simulink model "IEEE13_DVR_DSTATCOM_PV_Wind"  (R2022a)
settings: Solver=ode4  StartTime=0.0  StopTime=1.0  FixedStep=Ts  MaxStep=1e-4  RelTol=1e-4
InitFcn:
  | a=1; % Loading Factor
  | Ts=50e-6;
  | % phase to sequence conversion of RXB matrices
  | c=1*exp(sqrt(-1)*(120*pi/180));
  | T=[1 1 1;1 c*c c;1 c c*c];
  | Tinv=1/3*[1 1 1;1 c c*c;1 c*c c];
  | 
  | % Simulation data for the IEEE 13 Node Test Feeder model
  | mi2km = 1.60934;%  miles to km conversion
  | ft2km = 0.0003048; % feet to km conversion
  | ms2F = 1*1e-6/(2*pi*60);% microsiemens to Farads conversion
  | 
  | 
  | %% Configuration 601
  | % Series Resitance and Reactance - ohm/mile
  | R_601 = [0.3465 0.1560 0.1580;0.1560 0.3375 0.1535;0.1580 0.1535 0.3414];
  | X_601 = [1.1079 0.5017 0.4236;0.5017 1.0478 0.3849;0.4236 0.3849 1.0348];
  | % charging susceptance - microsiemens/mile
  | B_601 = [6.2998 -1.9958 -1.2595;-1.9958 5.9597 -0.7417;-1.2595 -0.7417 5.6386];
  | 
  | R_601 = R_601/mi2km;
  | Rseq=Tinv*R_601*T;
  | R1_601=Rseq(2,2);R0_601=Rseq(1,1);
  | 
  | L_601 = (X_601/(2*pi*60))/mi2km;
  | Lseq=Tinv*L_601*T;
  | L1_601=Lseq(2,2);L0_601=Lseq(1,1);
  | 
  | C_601 =(B_601*ms2F)/mi2km;
  | Cseq=Tinv*C_601*T;
  | C1_601=Cseq(2,2);C0_601=Cseq(1,1);
  | 
  | %% Configuration 602 - series reactance - ohm/mile
  | R_602 = [0.7526 0.1580 0.1560;0.1580 0.7475 0.1535;0.1560 0.1535 0.7436];
  | X_602 = [1.1814 0.4236 0.5017;0.4236 1.1983 0.3849;0.5017 0.3849 1.2112];
  | % charging susceptance - microsiemens/mile
  | B_602 = [5.6990 -1.0817 -1.6905;-1.0817 5.1795 -0.6588;-1.6905 -0.6588 5.4246];
  | 
  | R_602 = R_602/mi2km;
  | Rseq=Tinv*R_602*T;
  | R1_602=Rseq(2,2);R0_602=Rseq(1,1);
  | 
  | L_602 = (X_602/(2*pi*60))/mi2km;
  | Lseq=Tinv*L_602*T;
  | L1_602=Lseq(2,2);L0_602=Lseq(1,1);
  | 
  | C_602 =(B_602*ms2F)/mi2km;
  | Cseq=Tinv*C_602*T;
  | C1_602=Cseq(2,2);C0_602=Cseq(1,1);
  | %% Configuration 603 - series reactance - ohm/mile
  | R_603 = [0 0 0;0 1.3294 0.2066;0 0.2066 1.3238];
  | X_603 = [0 0 0;0 1.3471 0.4591;0 0.4591 1.3569];
  | % charging susceptance - microsiemens/mile
  | B_603 = [0 0 0;0 4.7097 -0.8999;0 -0.8999 4.6658];
  | 
  | % convert for SPS
  | R_603 = R_603/mi2km;
  | Rseq=Tinv*R_603*T;
  | R1_603=Rseq(2,2);R0_603=Rseq(1,1);
  | 
  | ... (+71 lines)
undefined symbols (not defined in the file): find_system
libraries: spsGroundLib x48, spsSeriesRLCBranchLib x46, spsThreePhaseVIMeasurementLib x19, spsControlledVoltageSourceLib x15, spsThreePhaseSeriesRLCLoadLib x7, spsRMSLib x7, spsThreePhaseBreakerLib x6, spsVoltageMeasurementLib x6, spsOnDelayLib x6, spsThreePhasePISectionLineLib x5, spsSeriesRLCLoadLib x5, spsMutualInductanceLib x4
(part 2 of 4)

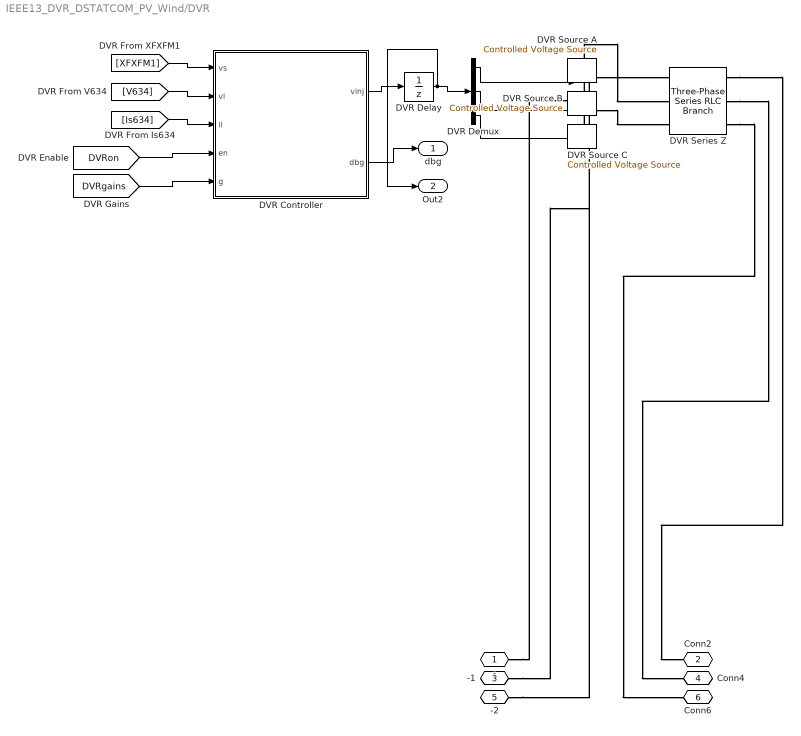
== system IEEE13_DVR_DSTATCOM_PV_Wind/DVR ==
  DVR Controller : MATLAB Function  TreatAsAtomicUnit=on
  DVR Delay : UnitDelay  SampleTime=-1  HasFrameUpgradeWarning=on
  DVR Demux : Demux  Outputs=3
  DVR Series Z : spsThreePhaseSeriesRLCBranchLib/Three-Phase Series RLC Branch  LConnTagsString=A|B|C  RConnTagsString=A|B|C  BranchType=RL  Resistance=2e-3  Inductance=60e-6  Capacitance=1e-6  Measurements=None
  DVR Source A : spsControlledVoltageSourceLib/Controlled Voltage Source  Initialize=off  Source_Type=AC  Amplitude=0  Phase=0  Frequency=0  Measurements=None
  DVR Source B : spsControlledVoltageSourceLib/Controlled Voltage Source  Initialize=off  Source_Type=AC  Amplitude=0  Phase=0  Frequency=0  Measurements=None
  DVR Source C : spsControlledVoltageSourceLib/Controlled Voltage Source  Initialize=off  Source_Type=AC  Amplitude=0  Phase=0  Frequency=0  Measurements=None
  - : PMIOPort  Side=Left
  Conn2 : PMIOPort  Port=2  Side=Right
  -1 : PMIOPort  Port=3  Side=Left
  Conn4 : PMIOPort  Port=4  Side=Right
  -2 : PMIOPort  Port=5  Side=Left
  Conn6 : PMIOPort  Port=6  Side=Right
  dbg : Outport
  Out2 : Outport  Port=2
  wires:
  DVR Demux/3 -> DVR Source C/1
  DVR Controller/1(vinj) -> DVR Delay/1
  DVR Delay/1 -> Out2/1, DVR Demux/1
  DVR Demux/2 -> DVR Source B/1
  [Is634] -> DVR Controller/3(il)
  [XFXFM1] -> DVR Controller/1(vs)
  DVR Demux/1 -> DVR Source A/1
  [V634] -> DVR Controller/2(vl)
  DVR Controller/2(dbg) -> dbg/1
  [DVRon] -> DVR Controller/4(en)
  [DVRgains] -> DVR Controller/5(g)
  connections:
  DVR Series Z/RConn2 -- Conn4/RConn1
  -2/RConn1 -- DVR Source C/LConn1
  DVR Series Z/RConn1 -- Conn2/RConn1
  DVR Source A/RConn1 -- DVR Series Z/LConn1
  DVR Source B/RConn1 -- DVR Series Z/LConn2
  DVR Source C/RConn1 -- DVR Series Z/LConn3
  -1/RConn1 -- DVR Source B/LConn1
  -/RConn1 -- DVR Source A/LConn1
  DVR Series Z/RConn3 -- Conn6/RConn1

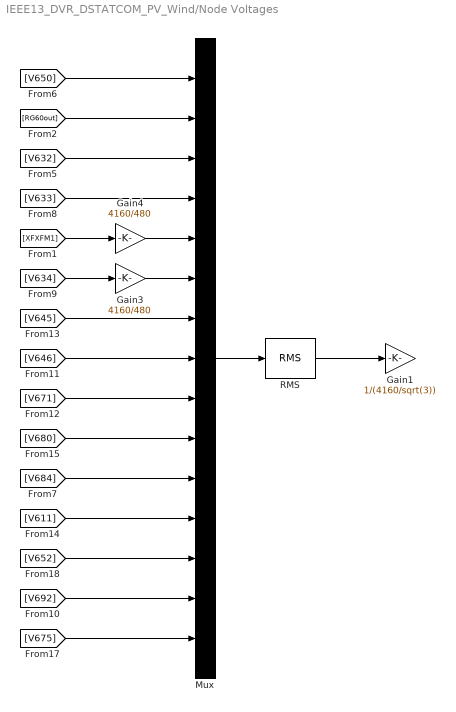
== system IEEE13_DVR_DSTATCOM_PV_Wind/Node Voltages ==
  Gain1 : Gain  Gain=1/(4160/sqrt(3))
  Gain3 : Gain  Gain=4160/480
  Gain4 : Gain  Gain=4160/480
  Mux : Mux  Inputs=15
  RMS : spsRMSLib/RMS  TrueRMS=on  Freq=60  RMSInit=120  Ts=0
  wires:
  RMS/1 -> Gain1/1
  Mux/1 -> RMS/1
  [V634] -> Gain3/1
  [V684] -> Mux/11
  [V675] -> Mux/15
  [V646] -> Mux/8
  [V633] -> Mux/4
  Gain3/1 -> Mux/6
  [XFXFM1] -> Gain4/1
  [V611] -> Mux/12
  [V632] -> Mux/3
  [V671] -> Mux/9
  [V680] -> Mux/10
  [V650] -> Mux/1
  [V652] -> Mux/13
  [RG60out] -> Mux/2
  [V692] -> Mux/14
  [V645] -> Mux/7
  Gain4/1 -> Mux/5

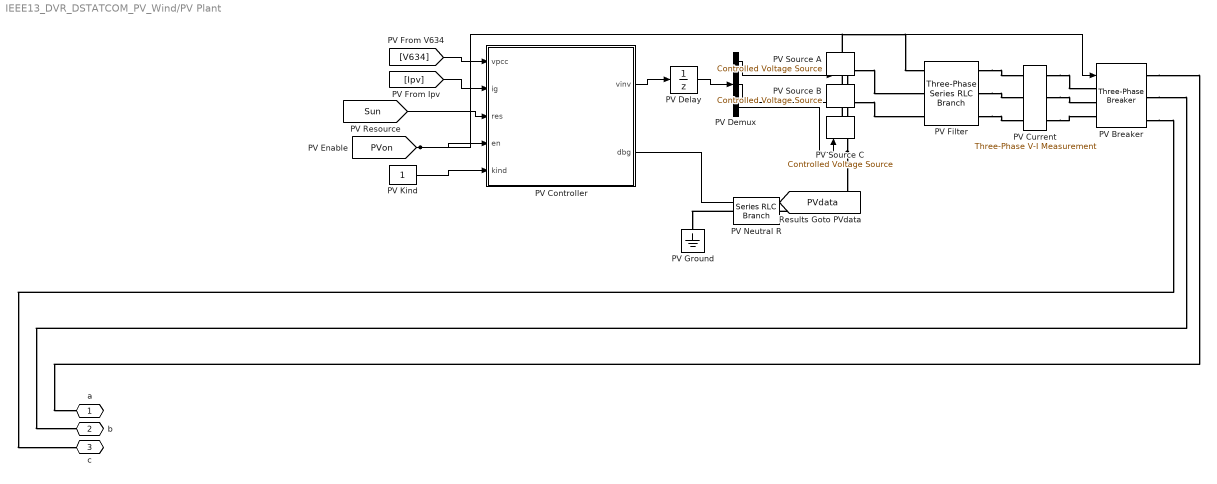
== system IEEE13_DVR_DSTATCOM_PV_Wind/PV Plant ==
  PV Breaker : spsThreePhaseBreakerLib/Three-Phase Breaker  InitialState=open  SwitchA=on  SwitchB=on  SwitchC=on  SwitchTimes=[0.2]  External=on  BreakerResistance=0.01  SnubberResistance=1e6  SnubberCapacitance=inf  Measurements=None
  PV Controller : MATLAB Function  TreatAsAtomicUnit=on
  PV Current : spsThreePhaseVIMeasurementLib/Three-Phase V-I Measurement  VoltageMeasurement=no  SetLabelV=off  LabelV=Vabc  Vpu=off  VpuLL=off  CurrentMeasurement=yes  SetLabelI=on  LabelI=Ipv  Ipu=off  Pbase=100e6  Vbase=500e3  OutputType=Complex  PhasorSimulation=off  PSBequivalent=0
  PV Delay : UnitDelay  SampleTime=-1  HasFrameUpgradeWarning=on
  PV Demux : Demux  Outputs=3
  PV Filter : spsThreePhaseSeriesRLCBranchLib/Three-Phase Series RLC Branch  LConnTagsString=A|B|C  RConnTagsString=A|B|C  BranchType=RL  Resistance=0.01*480^2/450e3  Inductance=0.1*480^2/450e3/(2*pi*60)  Capacitance=1e-6  Measurements=None
  PV Ground : spsGroundLib/Ground  LConnTagsString=a
  PV Kind : Constant  SampleTime=50e-6
  PV Neutral R : spsSeriesRLCBranchLib/Series RLC Branch  LConnTagsString=__new0  RConnTagsString=__new0  BranchType=R  Resistance=1e6  Inductance=1e-3  SetiL0=off  InitialCurrent=0  Capacitance=1e-6  Setx0=off  InitialVoltage=0  Measurements=None
  PV Source A : spsControlledVoltageSourceLib/Controlled Voltage Source  Initialize=off  Source_Type=AC  Amplitude=0  Phase=0  Frequency=0  Measurements=None
  PV Source B : spsControlledVoltageSourceLib/Controlled Voltage Source  Initialize=off  Source_Type=AC  Amplitude=0  Phase=0  Frequency=0  Measurements=None
  PV Source C : spsControlledVoltageSourceLib/Controlled Voltage Source  Initialize=off  Source_Type=AC  Amplitude=0  Phase=0  Frequency=0  Measurements=None
  a : PMIOPort  Side=Right
  b : PMIOPort  Port=2  Side=Right
  c : PMIOPort  Port=3  Side=Right
  tag scope: PVdata=global
  wires:
  [V634] -> PV Controller/1(vpcc)
  [Ipv] -> PV Controller/2(ig)
  PV Delay/1 -> PV Demux/1
  PV Kind/1 -> PV Controller/5(kind)
  PV Controller/2(dbg) -> [PVdata]
  PV Controller/1(vinv) -> PV Delay/1
  PV Demux/1 -> PV Source A/1
  PV Demux/3 -> PV Source C/1
  PV Demux/2 -> PV Source B/1
  [PVon] -> PV Controller/4(en), PV Breaker/1
  [Sun] -> PV Controller/3(res)
  connections:
  PV Source A/LConn1 -- PV Neutral R/RConn1 -- PV Source C/LConn1 -- PV Source B/LConn1
  PV Neutral R/LConn1 -- PV Ground/LConn1
  PV Filter/RConn1 -- PV Current/LConn1
  PV Source B/RConn1 -- PV Filter/LConn2
  PV Source C/RConn1 -- PV Filter/LConn3
  PV Filter/RConn2 -- PV Current/LConn2
  PV Filter/RConn3 -- PV Current/LConn3
  PV Current/RConn3 -- PV Breaker/LConn3
  PV Source A/RConn1 -- PV Filter/LConn1
  PV Current/RConn1 -- PV Breaker/LConn1
  PV Current/RConn2 -- PV Breaker/LConn2
  PV Breaker/RConn1 -- a/RConn1
  PV Breaker/RConn3 -- c/RConn1
  PV Breaker/RConn2 -- b/RConn1

== system IEEE13_DVR_DSTATCOM_PV_Wind/Regulator 1 ==
  Mux : Mux  Inputs=3
  Single Phase SVR_A : Subsystem  LoadFcn=find_system(gcs,'FollowLinks', 'on', 'LookUnderMasks', 'all');  mask(Single-Phase OLTC){pNom=5e6/3, fNom=60, vNom=4160/sqrt(3), ctRatio=700, ptRatio=20, DeltaU=0.00625, TapMinMax=[-16 16], InitialTap=-10, TapSelectionTime=0.2, RegulatorOn=on, Regulator=[122/120  2/120  0.2], Comp=[3 9]}
      mask prompts: pNom "Nominal Power (VA)"; fNom "Nominal Frequency (Hz)"; vNom "Nominal Voltage (Vrms)"; ctRatio "Primary CT Rating (A)"; ptRatio "PT Ratio"; DeltaU "Voltage Step Per Tap (pu)"; TapMinMax "Minimum and Maximum Tap Positions"; InitialTap "Initial Tap Position"; TapSelectionTime "Tap Selection Time (s)"; RegulatorOn "Voltage Regulator"; Regulator "Voltage Regulator [ Vref(pu) DeadBand(pu)  Delay(s)]"; Comp "Compensator Settings [R (V) X(V)]"
      mask help:
      | Models a single-phase On Load Tap Changer (OLTC). The single-phase primary of multi-tap winding is modeled with a Variable-Ratio Transformer block.
      |
      | The transformer voltage ratio U2/U1 (in pu) is given by:
      |                 U2/U1= 1/ (1+TapPosition*DeltaU)
      | Tap position 0 corresponds to nominal voltage ratio.
      |
      | When Voltage regulator is 'on',  voltage regulator asks for a tap change if:
      |                  abs(Vm-Vref)>DeadBand/2  during a time  t > Delay.
      |
      | where 'Vm' is voltage measured at regulating point and Vref is reference voltage.
      | With line drop compensation, Vm=Vsec-Isec(R+jX)
      mask init:
      | RegulatorVref=Regulator(1);
      | RegulatorDeadBand=Regulator(2);
      | RegulatorDelay=Regulator(3);
      | Rc=Comp(1);
      | Xc=Comp(2);
      mask TypeOptions RegulatorOn: off | on
      mask Callback RegulatorOn:
      | tempMaskVis=get_param(gcb,'MaskVisibilities');
      | if strcmp(get_param(gcb,'RegulatorOn'),'on')
      | 	tempMaskVis{11}='on';
      | 	set_param(gcb,'MaskVisibilities',tempMaskVis);
      | else
      | 	tempMaskVis{11}='off';
      | 	set_param(gcb,'MaskVisibilities',tempMaskVis);
      | end
      | if strcmp(get_param(gcb,'RegulatorOn'),'on')
      | 	tempMaskVis{12}='on';
      | 	set_param(gcb,'MaskVisibilities',tempMaskVis);
      | else
      | 	tempMaskVis{12}='off';
      | 	set_param(gcb,'MaskVisibilities',tempMaskVis);
      | end
      mask DialogControl Container8 Prompt: Setup
      mask DialogControl Container13 Prompt: Regulator Parameters
      mask Display:
      | color('blue');
      | r=50;x=40;y=80;
      | th = 0:pi/100:2*pi;
      | f = r * exp(j*th) + x+j*y;
      | plot(real(f), imag(f));
      | color('red');
      | plot([-10 90],[30,130])
      | plot([75 90],[125,130])
      | plot([85 90],[115,130])
      | color('black')
      | port_label('Lconn',1,'S');port_label('Rconn',1,'L');
  Single Phase SVR_B : Subsystem  LoadFcn=find_system(gcs,'FollowLinks', 'on', 'LookUnderMasks', 'all');  mask(Single-Phase OLTC){pNom=5e6/3, fNom=60, vNom=4160/sqrt(3), ctRatio=700, ptRatio=20, DeltaU=0.00625, TapMinMax=[-16 16], InitialTap=-8, TapSelectionTime=0.2, RegulatorOn=on, Regulator=[122/120  2/120  0.2], Comp=[3 9]}
      mask prompts: pNom "Nominal Power (VA)"; fNom "Nominal Frequency (Hz)"; vNom "Nominal Voltage (Vrms)"; ctRatio "Primary CT Rating (A)"; ptRatio "PT Ratio"; DeltaU "Voltage Step Per Tap (pu)"; TapMinMax "Minimum and Maximum Tap Positions"; InitialTap "Initial Tap Position"; TapSelectionTime "Tap Selection Time (s)"; RegulatorOn "Voltage Regulator"; Regulator "Voltage Regulator [ Vref(pu) DeadBand(pu)  Delay(s)]"; Comp "Compensator Settings [R (V) X(V)]"
      mask help:
      | Models a single-phase On Load Tap Changer (OLTC). The single-phase primary of multi-tap winding is modeled with a Variable-Ratio Transformer block.
      |
      | The transformer voltage ratio U2/U1 (in pu) is given by:
      |                 U2/U1= 1/ (1+TapPosition*DeltaU)
      | Tap position 0 corresponds to nominal voltage ratio.
      |
      | When Voltage regulator is 'on',  voltage regulator asks for a tap change if:
      |                  abs(Vm-Vref)>DeadBand/2  during a time  t > Delay.
      |
      | where 'Vm' is voltage measured at regulating point and Vref is reference voltage.
      | With line drop compensation, Vm=Vsec-Isec(R+jX)
      mask init:
      | RegulatorVref=Regulator(1);
      | RegulatorDeadBand=Regulator(2);
      | RegulatorDelay=Regulator(3);
      | Rc=Comp(1);
      | Xc=Comp(2);
      mask TypeOptions RegulatorOn: off | on
      mask Callback RegulatorOn:
      | tempMaskVis=get_param(gcb,'MaskVisibilities');
      | if strcmp(get_param(gcb,'RegulatorOn'),'on')
      | 	tempMaskVis{11}='on';
      | 	set_param(gcb,'MaskVisibilities',tempMaskVis);
      | else
      | 	tempMaskVis{11}='off';
      | 	set_param(gcb,'MaskVisibilities',tempMaskVis);
      | end
      | if strcmp(get_param(gcb,'RegulatorOn'),'on')
      | 	tempMaskVis{12}='on';
      | 	set_param(gcb,'MaskVisibilities',tempMaskVis);
      | else
      | 	tempMaskVis{12}='off';
      | 	set_param(gcb,'MaskVisibilities',tempMaskVis);
      | end
      mask DialogControl Container8 Prompt: Setup
      mask DialogControl Container13 Prompt: Regulator Parameters
      mask Display:
      | color('blue');
      | r=50;x=40;y=80;
      | th = 0:pi/100:2*pi;
      | f = r * exp(j*th) + x+j*y;
      | plot(real(f), imag(f));
      | color('red');
      | plot([-10 90],[30,130])
      | plot([75 90],[125,130])
      | plot([85 90],[115,130])
      | color('black')
      | port_label('Lconn',1,'S');port_label('Rconn',1,'L');
  Single Phase SVR_C : Subsystem  LoadFcn=find_system(gcs,'FollowLinks', 'on', 'LookUnderMasks', 'all');  mask(Single-Phase OLTC){pNom=5e6/3, fNom=60, vNom=4160/sqrt(3), ctRatio=700, ptRatio=20, DeltaU=0.00625, TapMinMax=[-16 16], InitialTap=-11, TapSelectionTime=0.2, RegulatorOn=on, Regulator=[122/120  2/120  0.2], Comp=[3 9]}
      mask prompts: pNom "Nominal Power (VA)"; fNom "Nominal Frequency (Hz)"; vNom "Nominal Voltage (Vrms)"; ctRatio "Primary CT Rating (A)"; ptRatio "PT Ratio"; DeltaU "Voltage Step Per Tap (pu)"; TapMinMax "Minimum and Maximum Tap Positions"; InitialTap "Initial Tap Position"; TapSelectionTime "Tap Selection Time (s)"; RegulatorOn "Voltage Regulator"; Regulator "Voltage Regulator [ Vref(pu) DeadBand(pu)  Delay(s)]"; Comp "Compensator Settings [R (V) X(V)]"
      mask help:
      | Models a single-phase On Load Tap Changer (OLTC). The single-phase primary of multi-tap winding is modeled with a Variable-Ratio Transformer block.
      |
      | The transformer voltage ratio U2/U1 (in pu) is given by:
      |                 U2/U1= 1/ (1+TapPosition*DeltaU)
      | Tap position 0 corresponds to nominal voltage ratio.
      |
      | When Voltage regulator is 'on',  voltage regulator asks for a tap change if:
      |                  abs(Vm-Vref)>DeadBand/2  during a time  t > Delay.
      |
      | where 'Vm' is voltage measured at regulating point and Vref is reference voltage.
      | With line drop compensation, Vm=Vsec-Isec(R+jX)
      mask init:
      | RegulatorVref=Regulator(1);
      | RegulatorDeadBand=Regulator(2);
      | RegulatorDelay=Regulator(3);
      | Rc=Comp(1);
      | Xc=Comp(2);
      mask TypeOptions RegulatorOn: off | on
      mask Callback RegulatorOn:
      | tempMaskVis=get_param(gcb,'MaskVisibilities');
      | if strcmp(get_param(gcb,'RegulatorOn'),'on')
      | 	tempMaskVis{11}='on';
      | 	set_param(gcb,'MaskVisibilities',tempMaskVis);
      | else
      | 	tempMaskVis{11}='off';
      | 	set_param(gcb,'MaskVisibilities',tempMaskVis);
      | end
      | if strcmp(get_param(gcb,'RegulatorOn'),'on')
      | 	tempMaskVis{12}='on';
      | 	set_param(gcb,'MaskVisibilities',tempMaskVis);
      | else
      | 	tempMaskVis{12}='off';
      | 	set_param(gcb,'MaskVisibilities',tempMaskVis);
      | end
      mask DialogControl Container8 Prompt: Setup
      mask DialogControl Container13 Prompt: Regulator Parameters
      mask Display:
      | color('blue');
      | r=50;x=40;y=80;
      | th = 0:pi/100:2*pi;
      | f = r * exp(j*th) + x+j*y;
      | plot(real(f), imag(f));
      | color('red');
      | plot([-10 90],[30,130])
      | plot([75 90],[125,130])
      | plot([85 90],[115,130])
      | color('black')
      | port_label('Lconn',1,'S');port_label('Rconn',1,'L');
  A : PMIOPort  Side=Left
  a : PMIOPort  Port=2  Side=Right
  B : PMIOPort  Port=3  Side=Left
  b : PMIOPort  Port=4  Side=Right
  C : PMIOPort  Port=5  Side=Left
  c : PMIOPort  Port=6  Side=Right
  Tap : Outport
  wires:
  Mux/1 -> Tap/1
  Single Phase SVR_C/1(Tap) -> Mux/3
  Single Phase SVR_B/1(Tap) -> Mux/2
  Single Phase SVR_A/1(Tap) -> Mux/1
  connections:
  Single Phase SVR_C/RConn1 -- c/RConn1
  Single Phase SVR_C/LConn1 -- C/RConn1
  Single Phase SVR_B/RConn1 -- b/RConn1
  Single Phase SVR_B/LConn1 -- B/RConn1
  Single Phase SVR_A/LConn1 -- A/RConn1
  Single Phase SVR_A/RConn1 -- a/RConn1

== system IEEE13_DVR_DSTATCOM_PV_Wind/Regulator Taps  ==
  note: Here the taps of the Voltage Regulator are on primary side of transformers unlike in Benchmark document where taps are considered on secondary of transformer. Therefore the values used are negative of what is used in Benchmark document. Also the direction of Tap Operation will be in opposite direction as compared to Regulator having taps on secondary side of transformer.
  Band Width : Constant  Value=2
  Band Width1 : Constant  Value=2
  Gain : Gain  Gain=1/2
  Gain2 : Gain  Gain=1/2
  Scope3 : Scope  NumInputPorts=5
  Sum : Sum  Inputs=|++
  Sum1 : Sum  Inputs=|+-
  Tap : Scope
  Vref : Constant  Value=122
  Vref1 : Constant  Value=122
  wires:
  [Rg1] -> Tap/1
  Vref/1 -> Sum/1
  Band Width/1 -> Gain/1
  Gain/1 -> Sum/2
  Gain2/1 -> Sum1/2
  Band Width1/1 -> Gain2/1
  Vref1/1 -> Sum1/1
  Sum/1 -> Scope3/1  "Upper Limit"
  [Vr1a] -> Scope3/2  "Vra"
  [Vr1b] -> Scope3/3  "Vrb"
  [Vr1c] -> Scope3/4  "Vrc"
  Sum1/1 -> Scope3/5  "Lower Limit"

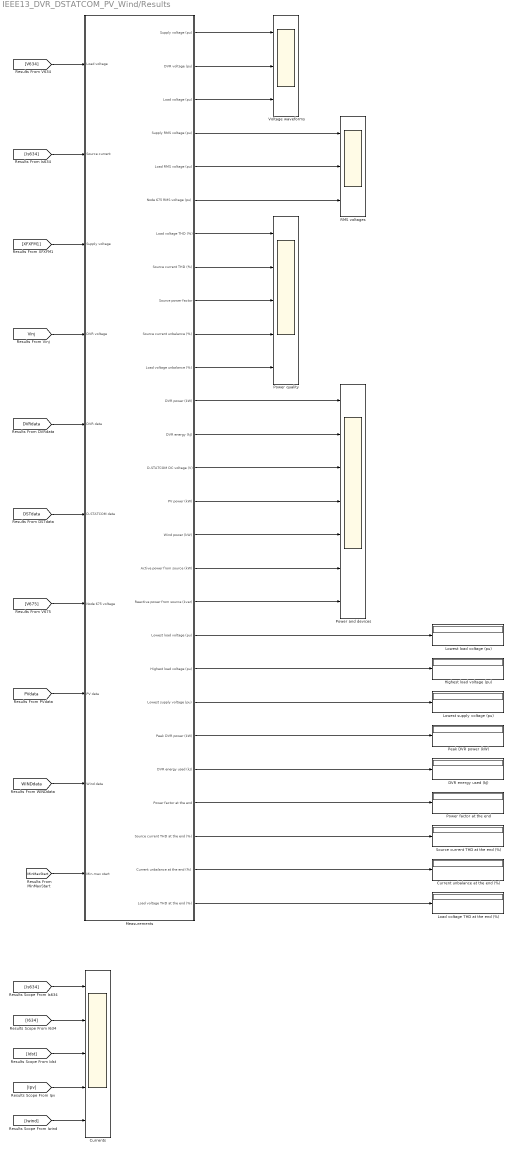
== system IEEE13_DVR_DSTATCOM_PV_Wind/Results ==
  Current unbalance at the end (%) : Display
      settings: Tag=results_panel
  Currents : Scope  NumInputPorts=5
      settings: Tag=results_panel
  DVR energy used (kJ) : Display
      settings: Tag=results_panel
  Highest load voltage (pu) : Display
      settings: Tag=results_panel
  Load voltage THD at the end (%) : Display
      settings: Tag=results_panel
  Lowest load voltage (pu) : Display
      settings: Tag=results_panel
  Lowest supply voltage (pu) : Display
      settings: Tag=results_panel
  Measurements : Subsystem  Tag=results_panel
  Peak DVR power (kW) : Display
      settings: Tag=results_panel
  Power and devices : Scope  NumInputPorts=7
      settings: Tag=results_panel
  Power factor at the end : Display
      settings: Tag=results_panel
  Power quality : Scope  NumInputPorts=5
      settings: Tag=results_panel
  RMS voltages : Scope  NumInputPorts=3
      settings: Tag=results_panel
  Source current THD at the end (%) : Display
      settings: Tag=results_panel
  Voltage waveforms : Scope  NumInputPorts=3
      settings: Tag=results_panel
  wires:
  Measurements/22(Peak DVR power (kW)) -> Peak DVR power (kW)/1
  [Idst] -> Currents/3
  Measurements/10(Source current unbalance (%)) -> Power quality/4
  [Is634] -> Currents/1
  Measurements/3(Load voltage (pu)) -> Voltage waveforms/3
  Measurements/19(Lowest load voltage (pu)) -> Lowest load voltage (pu)/1
  [WINDdata] -> Measurements/9(Wind data)
  Measurements/27(Load voltage THD at the end (%)) -> Load voltage THD at the end (%)/1
  Measurements/26(Current unbalance at the end (%)) -> Current unbalance at the end (%)/1
  [I634] -> Currents/2
  Measurements/2(DVR voltage (pu)) -> Voltage waveforms/2
  Measurements/14(D-STATCOM DC voltage (V)) -> Power and devices/3
  Measurements/16(Wind power (kW)) -> Power and devices/5
  Measurements/11(Load voltage unbalance (%)) -> Power quality/5
  Measurements/25(Source current THD at the end (%)) -> Source current THD at the end (%)/1
  [Vinj] -> Measurements/4(DVR voltage)
  Measurements/4(Supply RMS voltage (pu)) -> RMS voltages/1
  Measurements/13(DVR energy (kJ)) -> Power and devices/2
  Measurements/12(DVR power (kW)) -> Power and devices/1
  Measurements/24(Power factor at the end) -> Power factor at the end/1
  [Ipv] -> Currents/4
  Measurements/8(Source current THD (%)) -> Power quality/2
  Measurements/7(Load voltage THD (%)) -> Power quality/1
  Measurements/18(Reactive power from source (kvar)) -> Power and devices/7
  Measurements/20(Highest load voltage (pu)) -> Highest load voltage (pu)/1
  Measurements/6(Node 675 RMS voltage (pu)) -> RMS voltages/3
  Measurements/15(PV power (kW)) -> Power and devices/4
  Measurements/23(DVR energy used (kJ)) -> DVR energy used (kJ)/1
  [DVRdata] -> Measurements/5(DVR data)
  [Iwind] -> Currents/5
  Measurements/21(Lowest supply voltage (pu)) -> Lowest supply voltage (pu)/1
  Measurements/17(Active power from source (kW)) -> Power and devices/6
  Measurements/9(Source power factor) -> Power quality/3
  [Is634] -> Measurements/2(Source current)
  [PVdata] -> Measurements/8(PV data)
  Measurements/1(Supply voltage (pu)) -> Voltage waveforms/1
  [V675] -> Measurements/7(Node 675 voltage)
  Measurements/5(Load RMS voltage (pu)) -> RMS voltages/2
  [V634] -> Measurements/1(Load voltage)
  [DSTdata] -> Measurements/6(D-STATCOM data)
  [MinMaxStart] -> Measurements/10(Min-max start)
  [XFXFM1] -> Measurements/3(Supply voltage)

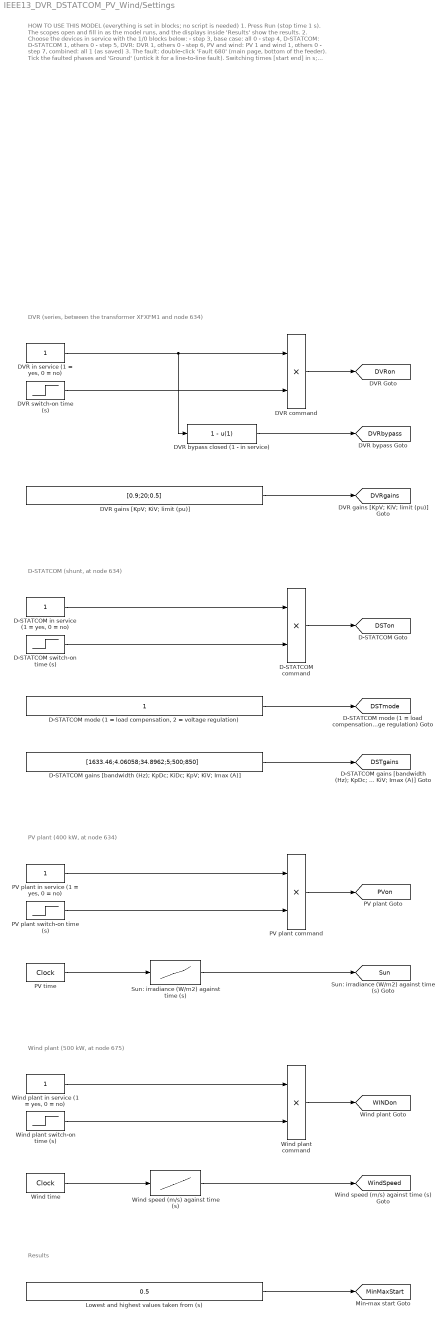
== system IEEE13_DVR_DSTATCOM_PV_Wind/Settings ==
  note: HOW TO USE THIS MODEL (everything is set in blocks; no script is needed)
      |
      | 1. Press Run (stop time 1 s). The scopes open and fill in as the model runs, and
      |    the displays inside 'Results' show the results.
      | 2. Choose the devices in service with the 1/0 blocks below:
      |    - step 3, base case: all 0
      |    - step 4, D-STATCOM: D-STATCOM 1, others 0
      |    - step 5, DVR: DVR 1, others 0
      |    - step 6, PV and wind: PV 1 and wind 1, others 0
      |    - step 7, combined: all 1 (as saved)
      | 3. The fault: double-click 'Fault 680' (main page, bottom of the feeder). Tick the faulted
      |    phases and 'Ground' (untick it for a line-to-line fault). Switching times
      |    [start end] in s; [100 100.1] means no fault. Saved: phase A to ground,
      |    0.6 to 0.8 s.
      | 4. The rectifier load: 'NL Breaker' (main page, next to node 634), switching time = when it
      |    connects (100 = never). Saved: 0.3 s.
      | 5. Gains: saved are the PSO gains. The hand-tuned gains of steps 4 and 5 are
      |    D-STATCOM [1500; 1; 15; 5; 500; 850] and DVR [0.2; 200; 0.5].
      | 6. Sun and wind: double-click the tables to give the irradiance or wind speed
      |    at chosen times, for example a cloud from 0.5 s.
      |
      | To compare runs, for example with and without a device: Simulation tab >
      | Data Inspector. Every run is kept there and the results can be overlaid.
      | Lowest and highest values are taken from 0.5 s on (last block on this page).
  note: Wind plant (500 kW, at node 675)
  note: PV plant (400 kW, at node 634)
  note: D-STATCOM (shunt, at node 634)
  note: DVR (series, between the transformer XFXFM1 and node 634)
  note: Results
  D-STATCOM command : Product
  D-STATCOM gains [bandwidth (Hz); KpDc; KiDc; KpV; KiV; Imax (A)] : Constant  Value=[1633.46;4.06058;34.8962;5;500;850]  SampleTime=50e-6
  "D-STATCOM in service (1 = yes, 0 = no)" : Constant
  "D-STATCOM mode (1 = load compensation, 2 = voltage regulation)" : Constant  SampleTime=50e-6
  D-STATCOM switch-on time (s) : Step  Time=0.4  SampleTime=50e-6
  DVR bypass closed (1 - in service) : Fcn  Expr=1 - u(1)
  DVR command : Product
  DVR gains [KpV; KiV; limit (pu)] : Constant  Value=[0.9;20;0.5]  SampleTime=50e-6
  "DVR in service (1 = yes, 0 = no)" : Constant
  DVR switch-on time (s) : Step  Time=0.4  SampleTime=50e-6
  Lowest and highest values taken from (s) : Constant  Tag=results_panel  Value=0.5
  PV plant command : Product
  "PV plant in service (1 = yes, 0 = no)" : Constant
  PV plant switch-on time (s) : Step  Time=0.2  SampleTime=50e-6
  PV time : DigitalClock  SampleTime=50e-6
  Sun: irradiance (W/m2) against time (s) : Lookup_n-D  NumberOfTableDimensions=1  BreakpointsForDimension1=[0 100]  Table=[1000 1000]  ExtrapMethod=Clip  InternalRulePriority=Speed  RndMeth=Simplest
  Wind plant command : Product
  "Wind plant in service (1 = yes, 0 = no)" : Constant
  Wind plant switch-on time (s) : Step  Time=0.2  SampleTime=50e-6
  Wind speed (m/s) against time (s) : Lookup_n-D  NumberOfTableDimensions=1  BreakpointsForDimension1=[0 100]  Table=[12 12]  ExtrapMethod=Clip  InternalRulePriority=Speed  RndMeth=Simplest
  Wind time : DigitalClock  SampleTime=50e-6
  tag scope: DSTgains=global, DSTmode=global, DSTon=global, DVRbypass=global, DVRgains=global, DVRon=global, MinMaxStart=global, PVon=global, Sun=global, WINDon=global, WindSpeed=global
  wires:
  Lowest and highest values taken from (s)/1 -> [MinMaxStart]
  D-STATCOM command/1 -> [DSTon]
  "D-STATCOM in service (1 = yes, 0 = no)"/1 -> D-STATCOM command/1
  PV plant switch-on time (s)/1 -> PV plant command/2
  DVR gains [KpV; KiV; limit (pu)]/1 -> [DVRgains]
  "DVR in service (1 = yes, 0 = no)"/1 -> DVR command/1, DVR bypass closed (1 - in service)/1
  D-STATCOM gains [bandwidth (Hz); KpDc; KiDc; KpV; KiV; Imax (A)]/1 -> [DSTgains]
  "D-STATCOM mode (1 = load compensation, 2 = voltage regulation)"/1 -> [DSTmode]
  Wind plant command/1 -> [WINDon]
  D-STATCOM switch-on time (s)/1 -> D-STATCOM command/2
  DVR switch-on time (s)/1 -> DVR command/2
  "PV plant in service (1 = yes, 0 = no)"/1 -> PV plant command/1
  PV time/1 -> Sun: irradiance (W/m2) against time (s)/1
  Sun: irradiance (W/m2) against time (s)/1 -> [Sun]
  DVR command/1 -> [DVRon]
  Wind plant switch-on time (s)/1 -> Wind plant command/2
  "Wind plant in service (1 = yes, 0 = no)"/1 -> Wind plant command/1
  DVR bypass closed (1 - in service)/1 -> [DVRbypass]
  Wind speed (m/s) against time (s)/1 -> [WindSpeed]
  PV plant command/1 -> [PVon]
  Wind time/1 -> Wind speed (m/s) against time (s)/1

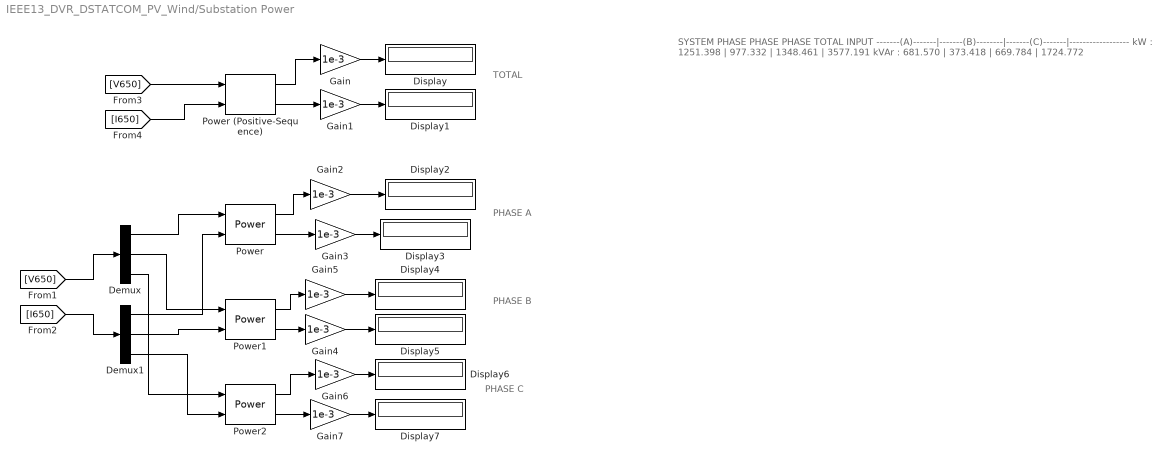
== system IEEE13_DVR_DSTATCOM_PV_Wind/Substation Power ==
  note: SYSTEM PHASE PHASE PHASE TOTAL
      | INPUT -------(A)-------|-------(B)--------|-------(C)-------|------------------
      | kW : 1251.398 | 977.332 | 1348.461 | 3577.191
      | kVAr : 681.570 | 373.418 | 669.784 | 1724.772
  note: PHASE A
  note: PHASE C
  note: PHASE B
  note: TOTAL
  Demux : Demux  Outputs=3
  Demux1 : Demux  Outputs=3
  Display{,1..7} (8 alike) : Display
  Gain{,1..7} (8 alike) : Gain  Gain=1e-3
  Power : spsPowerLib/Power  Freq=60  Vinit=[1, 0]  Iinit=[1, 0]  Ts=0
  Power (Positive-Sequence) : spsPowerPositiveSequenceLib/Power (Positive-Sequence)  Freq=60  Vinit=[0, 0]  Iinit=[0, 0]  Ts=Ts
  Power1 : spsPowerLib/Power  Freq=60  Vinit=[1, 0]  Iinit=[1, 0]  Ts=0
  Power2 : spsPowerLib/Power  Freq=60  Vinit=[1, 0]  Iinit=[1, 0]  Ts=0
  wires:
  [I650] -> Power (Positive-Sequence)/2
  [V650] -> Power (Positive-Sequence)/1
  Power (Positive-Sequence)/1 -> Gain/1
  Power (Positive-Sequence)/2 -> Gain1/1
  [V650] -> Demux/1
  [I650] -> Demux1/1
  Demux/1 -> Power/1
  Demux1/1 -> Power/2
  Demux/2 -> Power1/1
  Demux1/2 -> Power1/2
  Demux/3 -> Power2/1
  Demux1/3 -> Power2/2
  Power/1 -> Gain2/1
  Power/2 -> Gain3/1
  Power1/1 -> Gain5/1
  Power1/2 -> Gain4/1
  Power2/1 -> Gain6/1
  Power2/2 -> Gain7/1
  Gain/1 -> Display/1
  Gain1/1 -> Display1/1
  Gain2/1 -> Display2/1
  Gain3/1 -> Display3/1
  Gain4/1 -> Display5/1
  Gain5/1 -> Display4/1
  Gain6/1 -> Display6/1
  Gain7/1 -> Display7/1

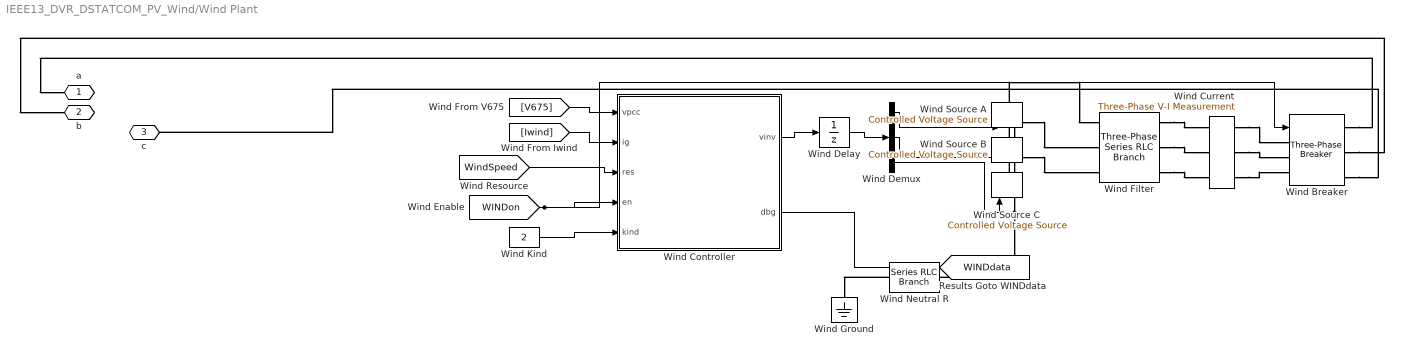
== system IEEE13_DVR_DSTATCOM_PV_Wind/Wind Plant ==
  Wind Breaker : spsThreePhaseBreakerLib/Three-Phase Breaker  InitialState=open  SwitchA=on  SwitchB=on  SwitchC=on  SwitchTimes=[0.2]  External=on  BreakerResistance=0.01  SnubberResistance=1e6  SnubberCapacitance=inf  Measurements=None
  Wind Controller : MATLAB Function  TreatAsAtomicUnit=on
  Wind Current : spsThreePhaseVIMeasurementLib/Three-Phase V-I Measurement  VoltageMeasurement=no  SetLabelV=off  LabelV=Vabc  Vpu=off  VpuLL=off  CurrentMeasurement=yes  SetLabelI=on  LabelI=Iwind  Ipu=off  Pbase=100e6  Vbase=500e3  OutputType=Complex  PhasorSimulation=off  PSBequivalent=0
  Wind Delay : UnitDelay  SampleTime=-1  HasFrameUpgradeWarning=on
  Wind Demux : Demux  Outputs=3
  Wind Filter : spsThreePhaseSeriesRLCBranchLib/Three-Phase Series RLC Branch  LConnTagsString=A|B|C  RConnTagsString=A|B|C  BranchType=RL  Resistance=0.01*4160^2/550e3  Inductance=0.1*4160^2/550e3/(2*pi*60)  Capacitance=1e-6  Measurements=None
  Wind Ground : spsGroundLib/Ground  LConnTagsString=a
  Wind Kind : Constant  Value=2  SampleTime=50e-6
  Wind Neutral R : spsSeriesRLCBranchLib/Series RLC Branch  LConnTagsString=__new0  RConnTagsString=__new0  BranchType=R  Resistance=1e6  Inductance=1e-3  SetiL0=off  InitialCurrent=0  Capacitance=1e-6  Setx0=off  InitialVoltage=0  Measurements=None
  Wind Source A : spsControlledVoltageSourceLib/Controlled Voltage Source  Initialize=off  Source_Type=AC  Amplitude=0  Phase=0  Frequency=0  Measurements=None
  Wind Source B : spsControlledVoltageSourceLib/Controlled Voltage Source  Initialize=off  Source_Type=AC  Amplitude=0  Phase=0  Frequency=0  Measurements=None
  Wind Source C : spsControlledVoltageSourceLib/Controlled Voltage Source  Initialize=off  Source_Type=AC  Amplitude=0  Phase=0  Frequency=0  Measurements=None
  a : PMIOPort  Side=Right
  b : PMIOPort  Port=2  Side=Right
  c : PMIOPort  Port=3  Side=Right
  tag scope: WINDdata=global
  wires:
  Wind Controller/1(vinv) -> Wind Delay/1
  Wind Delay/1 -> Wind Demux/1
  [Iwind] -> Wind Controller/2(ig)
  Wind Controller/2(dbg) -> [WINDdata]
  Wind Demux/1 -> Wind Source A/1
  Wind Demux/3 -> Wind Source C/1
  [V675] -> Wind Controller/1(vpcc)
  Wind Kind/1 -> Wind Controller/5(kind)
  Wind Demux/2 -> Wind Source B/1
  [WINDon] -> Wind Controller/4(en), Wind Breaker/1
  [WindSpeed] -> Wind Controller/3(res)
  connections:
  Wind Current/RConn2 -- Wind Breaker/LConn2
  Wind Filter/RConn2 -- Wind Current/LConn2
  Wind Source A/RConn1 -- Wind Filter/LConn1
  Wind Source A/LConn1 -- Wind Neutral R/RConn1 -- Wind Source C/LConn1 -- Wind Source B/LConn1
  Wind Source B/RConn1 -- Wind Filter/LConn2
  Wind Current/RConn1 -- Wind Breaker/LConn1
  Wind Breaker/RConn1 -- a/RConn1
  Wind Filter/RConn3 -- Wind Current/LConn3
  Wind Source C/RConn1 -- Wind Filter/LConn3
  Wind Filter/RConn1 -- Wind Current/LConn1
  Wind Neutral R/LConn1 -- Wind Ground/LConn1
  Wind Breaker/RConn3 -- c/RConn1
  Wind Current/RConn3 -- Wind Breaker/LConn3
  Wind Breaker/RConn2 -- b/RConn1

== system IEEE13_DVR_DSTATCOM_PV_Wind/Regulator 1/Single Phase SVR_A ==
  Line Drop Compensator : Subsystem
  Transformer with Taps : Subsystem
  Voltage Regulator Control : Subsystem
  S : PMIOPort  Tag=PMCPort  Side=Left
  L : PMIOPort  Tag=PMCPort  Port=2  Side=Right
  Tap : Outport  VectorParamsAs1DForOutWhenUnconnected=off
  tag scope: Vr1a=global
  wires:
  Line Drop Compensator/1(Vm) -> Voltage Regulator Control/1(Vm), [Vr1a]
  Voltage Regulator Control/2(Tap) -> Tap/1
  Voltage Regulator Control/1(N) -> Transformer with Taps/1(N)
  Transformer with Taps/1(Isec) -> Line Drop Compensator/1(Isec)
  Transformer with Taps/2(Vsec) -> Line Drop Compensator/2(Vsec)
  connections:
  Transformer with Taps/RConn1 -- L/RConn1
  S/RConn1 -- Transformer with Taps/LConn1

== system IEEE13_DVR_DSTATCOM_PV_Wind/Regulator 1/Single Phase SVR_B ==
  Line Drop Compensator : Subsystem
  Transformer with Taps : Subsystem
  Voltage Regulator Control : Subsystem
  S : PMIOPort  Tag=PMCPort  Side=Left
  L : PMIOPort  Tag=PMCPort  Port=2  Side=Right
  Tap : Outport  VectorParamsAs1DForOutWhenUnconnected=off
  tag scope: Vr1b=global
  wires:
  Transformer with Taps/2(Vsec) -> Line Drop Compensator/2(Vsec)
  Transformer with Taps/1(Isec) -> Line Drop Compensator/1(Isec)
  Voltage Regulator Control/1(N) -> Transformer with Taps/1(N)
  Voltage Regulator Control/2(Tap) -> Tap/1
  Line Drop Compensator/1(Vm) -> [Vr1b], Voltage Regulator Control/1(Vm)
  connections:
  S/RConn1 -- Transformer with Taps/LConn1
  Transformer with Taps/RConn1 -- L/RConn1

== system IEEE13_DVR_DSTATCOM_PV_Wind/Regulator 1/Single Phase SVR_C ==
  Line Drop Compensator : Subsystem
  Transformer with Taps : Subsystem
  Voltage Regulator Control : Subsystem
  S : PMIOPort  Tag=PMCPort  Side=Left
  L : PMIOPort  Tag=PMCPort  Port=2  Side=Right
  Tap : Outport  VectorParamsAs1DForOutWhenUnconnected=off
  tag scope: Vr1c=global
  wires:
  Line Drop Compensator/1(Vm) -> Voltage Regulator Control/1(Vm), [Vr1c]
  Voltage Regulator Control/2(Tap) -> Tap/1
  Voltage Regulator Control/1(N) -> Transformer with Taps/1(N)
  Transformer with Taps/1(Isec) -> Line Drop Compensator/1(Isec)
  Transformer with Taps/2(Vsec) -> Line Drop Compensator/2(Vsec)
  connections:
  Transformer with Taps/RConn1 -- L/RConn1
  S/RConn1 -- Transformer with Taps/LConn1

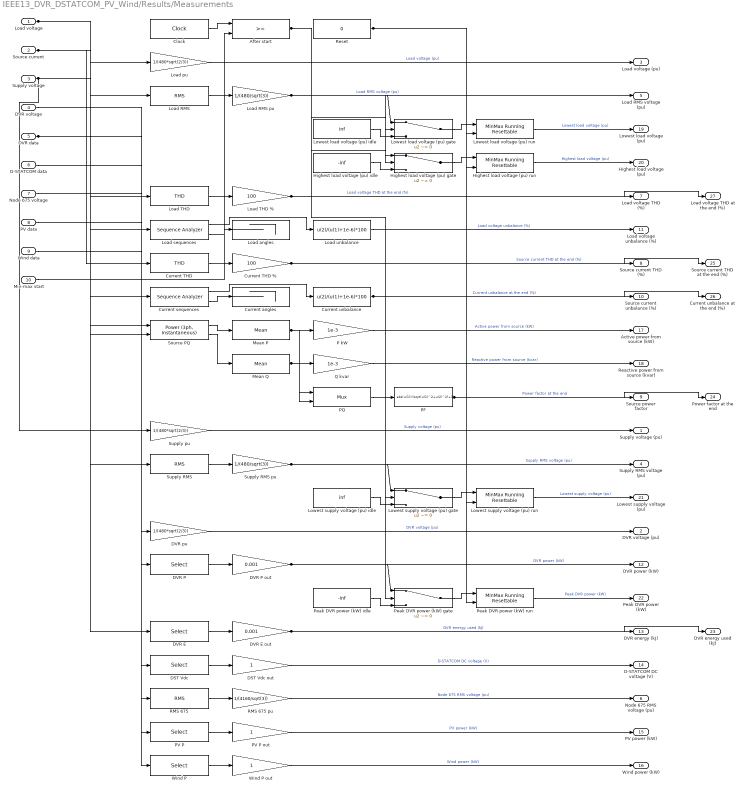
== system IEEE13_DVR_DSTATCOM_PV_Wind/Results/Measurements ==
  Load voltage : Inport
  Source current : Inport  Port=2
  Supply voltage : Inport  Port=3
  DVR voltage : Inport  Port=4
  DVR data : Inport  Port=5
  D-STATCOM data : Inport  Port=6
  Node 675 voltage : Inport  Port=7
  PV data : Inport  Port=8
  Wind data : Inport  Port=9
  Min-max start : Inport  Port=10
  After start : RelationalOperator  OutDataTypeStr=boolean  RndMeth=Simplest  InputSameDT=off
  Clock : DigitalClock  SampleTime=50e-6
  Current THD : spsTHDLib/THD  Freq=60  Ts=50e-6
  Current THD % : Gain  Gain=100
  Current angles : Terminator
  Current sequences : spsSequenceAnalyzerLib/Sequence Analyzer  Freq=60  n=1  seq=Positive Negative Zero  InInit=[1, 0]  Ts=50e-6
  Current unbalance : Fcn  Expr=u(2)/(u(1)+1e-6)*100
  DST Vdc : Selector  InputPortWidth=8  IndexOptions=Index vector (dialog)  Indices=1  OutputSizes=1
  DST Vdc out : Gain
  DVR E : Selector  InputPortWidth=8  IndexOptions=Index vector (dialog)  Indices=2  OutputSizes=1
  DVR E out : Gain  Gain=0.001
  DVR P : Selector  InputPortWidth=8  IndexOptions=Index vector (dialog)  Indices=1  OutputSizes=1
  DVR P out : Gain  Gain=0.001
  DVR pu : Gain  Gain=1/(480*sqrt(2/3))
  Highest load voltage (pu) gate : Switch  Criteria=u2 ~= 0  SaturateOnIntegerOverflow=off  InputSameDT=off
  Highest load voltage (pu) idle : Constant  Value=-inf
  Highest load voltage (pu) run : simulink/Math Operations/MinMax Running Resettable  Function=max  vinit=-inf
  Load RMS : spsRMSLib/RMS  TrueRMS=on  Freq=60  RMSInit=480/sqrt(3)  Ts=50e-6
  Load RMS pu : Gain  Gain=1/(480/sqrt(3))
  Load THD : spsTHDLib/THD  Freq=60  Ts=50e-6
  Load THD % : Gain  Gain=100
  Load angles : Terminator
  Load pu : Gain  Gain=1/(480*sqrt(2/3))
  Load sequences : spsSequenceAnalyzerLib/Sequence Analyzer  Freq=60  n=1  seq=Positive Negative Zero  InInit=[1, 0]  Ts=50e-6
  Load unbalance : Fcn  Expr=u(2)/(u(1)+1e-6)*100
  Lowest load voltage (pu) gate : Switch  Criteria=u2 ~= 0  SaturateOnIntegerOverflow=off  InputSameDT=off
  Lowest load voltage (pu) idle : Constant  Value=inf
  Lowest load voltage (pu) run : simulink/Math Operations/MinMax Running Resettable  Function=min  vinit=inf
  Lowest supply voltage (pu) gate : Switch  Criteria=u2 ~= 0  SaturateOnIntegerOverflow=off  InputSameDT=off
  Lowest supply voltage (pu) idle : Constant  Value=inf
  Lowest supply voltage (pu) run : simulink/Math Operations/MinMax Running Resettable  Function=min  vinit=inf
  Mean P : spsMeanLib/Mean  Freq=60  Vinit=0  Ts=50e-6
  Mean Q : spsMeanLib/Mean  Freq=60  Vinit=0  Ts=50e-6
  P kW : Gain  Gain=1e-3
  PF : Fcn  Expr=abs(u(1))/(sqrt(u(1)^2+u(2)^2)+1)
  PQ : Mux  Inputs=2
  PV P : Selector  InputPortWidth=8  IndexOptions=Index vector (dialog)  Indices=2  OutputSizes=1
  PV P out : Gain
  Peak DVR power (kW) gate : Switch  Criteria=u2 ~= 0  SaturateOnIntegerOverflow=off  InputSameDT=off
  Peak DVR power (kW) idle : Constant  Value=-inf
  Peak DVR power (kW) run : simulink/Math Operations/MinMax Running Resettable  Function=max  vinit=-inf
  Q kvar : Gain  Gain=1e-3
  RMS 675 : spsRMSLib/RMS  TrueRMS=on  Freq=60  RMSInit=4160/sqrt(3)  Ts=50e-6
  RMS 675 pu : Gain  Gain=1/(4160/sqrt(3))
  Reset : Constant  Value=0
  Source PQ : spsPower3phInstantaneousLib/Power (3ph, Instantaneous)
  Supply RMS : spsRMSLib/RMS  TrueRMS=on  Freq=60  RMSInit=480/sqrt(3)  Ts=50e-6
  Supply RMS pu : Gain  Gain=1/(480/sqrt(3))
  Supply pu : Gain  Gain=1/(480*sqrt(2/3))
  Wind P : Selector  InputPortWidth=8  IndexOptions=Index vector (dialog)  Indices=2  OutputSizes=1
  Wind P out : Gain
  Supply voltage (pu) : Outport
  DVR voltage (pu) : Outport  Port=2
  Load voltage (pu) : Outport  Port=3
  Supply RMS voltage (pu) : Outport  Port=4
  Load RMS voltage (pu) : Outport  Port=5
  Node 675 RMS voltage (pu) : Outport  Port=6
  Load voltage THD (%) : Outport  Port=7
  Source current THD (%) : Outport  Port=8
  Source power factor : Outport  Port=9
  Source current unbalance (%) : Outport  Port=10
  Load voltage unbalance (%) : Outport  Port=11
  DVR power (kW) : Outport  Port=12
  DVR energy (kJ) : Outport  Port=13
  D-STATCOM DC voltage (V) : Outport  Port=14
  PV power (kW) : Outport  Port=15
  Wind power (kW) : Outport  Port=16
  Active power from source (kW) : Outport  Port=17
  Reactive power from source (kvar) : Outport  Port=18
  Lowest load voltage (pu) : Outport  Port=19
  Highest load voltage (pu) : Outport  Port=20
  Lowest supply voltage (pu) : Outport  Port=21
  Peak DVR power (kW) : Outport  Port=22
  DVR energy used (kJ) : Outport  Port=23
  Power factor at the end : Outport  Port=24
  Source current THD at the end (%) : Outport  Port=25
  Current unbalance at the end (%) : Outport  Port=26
  Load voltage THD at the end (%) : Outport  Port=27
  wires:
  Clock/1 -> After start/1
  Min-max start/1 -> After start/2
  Load voltage/1 -> Load pu/1, Load RMS/1, Load THD/1, Load sequences/1, Source PQ/1
  Load pu/1 -> Load voltage (pu)/1  "Load voltage (pu)"
  Load RMS/1 -> Load RMS pu/1
  Load RMS pu/1 -> Load RMS voltage (pu)/1, Lowest load voltage (pu) gate/1, Highest load voltage (pu) gate/1  "Load RMS voltage (pu)"
  After start/1 -> Lowest load voltage (pu) gate/2, Highest load voltage (pu) gate/2, Lowest supply voltage (pu) gate/2, Peak DVR power (kW) gate/2
  Lowest load voltage (pu) idle/1 -> Lowest load voltage (pu) gate/3
  Lowest load voltage (pu) gate/1 -> Lowest load voltage (pu) run/1
  Reset/1 -> Lowest load voltage (pu) run/2, Highest load voltage (pu) run/2, Lowest supply voltage (pu) run/2, Peak DVR power (kW) run/2
  Lowest load voltage (pu) run/1 -> Lowest load voltage (pu)/1  "Lowest load voltage (pu)"
  Highest load voltage (pu) idle/1 -> Highest load voltage (pu) gate/3
  Highest load voltage (pu) gate/1 -> Highest load voltage (pu) run/1
  Highest load voltage (pu) run/1 -> Highest load voltage (pu)/1  "Highest load voltage (pu)"
  Load THD/1 -> Load THD %/1
  Load THD %/1 -> Load voltage THD (%)/1, Load voltage THD at the end (%)/1  "Load voltage THD at the end (%)"
  Load sequences/2 -> Load angles/1
  Load sequences/1 -> Load unbalance/1
  Load unbalance/1 -> Load voltage unbalance (%)/1  "Load voltage unbalance (%)"
  Source current/1 -> Current THD/1, Current sequences/1, Source PQ/2
  Current THD/1 -> Current THD %/1
  Current THD %/1 -> Source current THD (%)/1, Source current THD at the end (%)/1  "Source current THD at the end (%)"
  Current sequences/2 -> Current angles/1
  Current sequences/1 -> Current unbalance/1
  Current unbalance/1 -> Source current unbalance (%)/1, Current unbalance at the end (%)/1  "Current unbalance at the end (%)"
  Source PQ/1 -> Mean P/1
  Mean P/1 -> P kW/1, PQ/1
  P kW/1 -> Active power from source (kW)/1  "Active power from source (kW)"
  Source PQ/2 -> Mean Q/1
  Mean Q/1 -> Q kvar/1, PQ/2
  Q kvar/1 -> Reactive power from source (kvar)/1  "Reactive power from source (kvar)"
  PQ/1 -> PF/1
  PF/1 -> Source power factor/1, Power factor at the end/1  "Power factor at the end"
  Supply voltage/1 -> Supply pu/1, Supply RMS/1
  Supply pu/1 -> Supply voltage (pu)/1  "Supply voltage (pu)"
  Supply RMS/1 -> Supply RMS pu/1
  Supply RMS pu/1 -> Supply RMS voltage (pu)/1, Lowest supply voltage (pu) gate/1  "Supply RMS voltage (pu)"
  Lowest supply voltage (pu) idle/1 -> Lowest supply voltage (pu) gate/3
  Lowest supply voltage (pu) gate/1 -> Lowest supply voltage (pu) run/1
  Lowest supply voltage (pu) run/1 -> Lowest supply voltage (pu)/1  "Lowest supply voltage (pu)"
  DVR voltage/1 -> DVR pu/1
  DVR pu/1 -> DVR voltage (pu)/1  "DVR voltage (pu)"
  DVR data/1 -> DVR P/1, DVR E/1
  DVR P/1 -> DVR P out/1
  DVR P out/1 -> DVR power (kW)/1, Peak DVR power (kW) gate/1  "DVR power (kW)"
  Peak DVR power (kW) idle/1 -> Peak DVR power (kW) gate/3
  Peak DVR power (kW) gate/1 -> Peak DVR power (kW) run/1
  Peak DVR power (kW) run/1 -> Peak DVR power (kW)/1  "Peak DVR power (kW)"
  DVR E/1 -> DVR E out/1
  DVR E out/1 -> DVR energy (kJ)/1, DVR energy used (kJ)/1  "DVR energy used (kJ)"
  D-STATCOM data/1 -> DST Vdc/1
  DST Vdc/1 -> DST Vdc out/1
  DST Vdc out/1 -> D-STATCOM DC voltage (V)/1  "D-STATCOM DC voltage (V)"
  Node 675 voltage/1 -> RMS 675/1
  RMS 675/1 -> RMS 675 pu/1
  RMS 675 pu/1 -> Node 675 RMS voltage (pu)/1  "Node 675 RMS voltage (pu)"
  PV data/1 -> PV P/1
  PV P/1 -> PV P out/1
  PV P out/1 -> PV power (kW)/1  "PV power (kW)"
  Wind data/1 -> Wind P/1
  Wind P/1 -> Wind P out/1
  Wind P out/1 -> Wind power (kW)/1  "Wind power (kW)"

== system IEEE13_DVR_DSTATCOM_PV_Wind/Regulator 1/Single Phase SVR_A/Line Drop Compensator ==
  note: Vm=Vsec-Isec(Rc+jXc)
  Isec : Inport
  Vsec : Inport  Port=2
  "        " : spsLinearTransformerLib/Linear Transformer  UNITS=SI  NominalPower=[pNom fNom]  winding1=[vNom/ptRatio 1e-7 1e-8]  winding2=[vNom/ptRatio 1e-7 1e-8]  ThreeWindings=off  winding3=[3.15e+005 0.7938 0.084225]  RmLm=[1e5 1e5]  Measurements=None  DataType=on
  "CTS  " : spsControlledCurrentSourceLib/Controlled Current Source  Initialize=on  Source_Type=AC  Amplitude=0  Phase=0  Frequency=0  Measurements=None
  "PTS  " : spsControlledVoltageSourceLib/Controlled Voltage Source  Initialize=on  Source_Type=AC  Amplitude=0  Phase=0  Frequency=0  Measurements=None
  RMS : spsRMSLib/RMS  TrueRMS=on  Freq=60  RMSInit=120  Ts=0
  Raux : spsSeriesRLCBranchLib/Series RLC Branch  LConnTagsString=__new0  RConnTagsString=__new0  BranchType=R  Resistance=1e3  Inductance=1.6 / (120*pi)  SetiL0=off  InitialCurrent=0  Capacitance=1e-6  Setx0=off  InitialVoltage=0  Measurements=None
  Rc+jXc : spsSeriesRLCBranchLib/Series RLC Branch  LConnTagsString=__new0  RConnTagsString=__new0  BranchType=RL  Resistance=Rc  Inductance=Xc / (2*pi*fNom)  SetiL0=off  InitialCurrent=0  Capacitance=1e-6  Setx0=off  InitialVoltage=0  Measurements=None
  VRelay : spsVoltageMeasurementLib/Voltage Measurement  PhasorSimulation=off  OutputType=Complex  PSBequivalent=0
  Vm : Outport
  wires:
  RMS/1 -> Vm/1
  VRelay/1 -> RMS/1
  Isec/1 -> "CTS  "/1
  Vsec/1 -> "PTS  "/1
  connections:
  "PTS  "/RConn1 -- "        "/RConn1
  "        "/RConn2 -- VRelay/LConn1
  Raux/LConn1 -- Rc+jXc/LConn1 -- "        "/LConn1 -- "CTS  "/RConn1
  Rc+jXc/RConn1 -- Raux/RConn1 -- "CTS  "/LConn1 -- "        "/LConn2
  VRelay/LConn2 -- "PTS  "/LConn1

== system IEEE13_DVR_DSTATCOM_PV_Wind/Regulator 1/Single Phase SVR_A/Transformer with Taps ==
  note: Vsec on Pt Ratio base
  note: Isec on CT Ratio base
  N : Inport
  "    " : Gain  Gain=1/ptRatio
  " 1" : Gain  Gain=1/ctRatio
  CT : spsCurrentMeasurementLib/Current Measurement  PhasorSimulation=off  OutputType=Complex  PSBequivalent=0
  Ground1 : spsGroundLib/Ground  LConnTagsString=a
  Ground2 : spsGroundLib/Ground  LConnTagsString=a
  Ground3 : spsGroundLib/Ground  LConnTagsString=a
  Memory : Memory
  Memory1 : Memory
  PT : spsVoltageMeasurementLib/Voltage Measurement  PhasorSimulation=off  OutputType=Complex  PSBequivalent=0
  "Variable-Ratio Transformer " : spsVariableRatioTransformerLib/Variable-Ratio Transformer
  rs : spsSeriesRLCBranchLib/Series RLC Branch  LConnTagsString=__new0  RConnTagsString=__new0  BranchType=R  Resistance=1e-6  Inductance=1e-3  SetiL0=off  InitialCurrent=0  Capacitance=1e-6  Setx0=off  InitialVoltage=0  Measurements=None
  L : PMIOPort  Tag=PMCPort  Side=Right
  S : PMIOPort  Port=2  Side=Left
  Isec : Outport
  Vsec : Outport  Port=2
  wires:
  "    "/1 -> Memory1/1
  PT/1 -> "    "/1
  CT/1 -> " 1"/1
  " 1"/1 -> Memory/1
  N/1 -> "Variable-Ratio Transformer "/1
  Memory1/1 -> Vsec/1
  Memory/1 -> Isec/1
  connections:
  PT/LConn2 -- Ground1/LConn1
  rs/RConn1 -- CT/LConn1 -- PT/LConn1
  CT/RConn1 -- L/RConn1
  "Variable-Ratio Transformer "/RConn1 -- rs/LConn1
  Ground3/LConn1 -- "Variable-Ratio Transformer "/LConn2
  Ground2/LConn1 -- "Variable-Ratio Transformer "/RConn2
  S/RConn1 -- "Variable-Ratio Transformer "/LConn1

== system IEEE13_DVR_DSTATCOM_PV_Wind/Regulator 1/Single Phase SVR_A/Voltage Regulator Control ==
  note: N= 1/ (1+TapPosition*DeltaU)
  Vm : Inport
  1 : Constant
  Constant : Constant  Value=RegulatorOn
  Constant5 : Constant
  Product : Product  Inputs=/*
  Sum : Sum
  Tap Changer Control : Subsystem  mask(Tap Changer Control){MinMaxTap=TapMinMax, InitialPosition=InitialTap, MecDelay=TapSelectionTime}
      mask prompts: MinMaxTap "Minimum and maximum tap number [ Min  Max ] :"; InitialPosition "Initial tap position"; MecDelay "Mechanical delay time"
      mask init:
      | if MecDelay<=0,
      | 	MecDelay=1/60;
      | end
  Voltage change per tap : Gain  Gain=DeltaU
  Voltage regulator : Subsystem  mask{Vref=RegulatorVref*120, DeadBand=RegulatorDeadBand*120, TimeDelay=RegulatorDelay}
      mask prompts: Vref "Vref (on 120v base)"; DeadBand "Deadband (on 120v base)"; TimeDelay "Time delay (s)"
  N : Outport
  Tap : Outport  Port=2
  wires:
  Vm/1 -> Voltage regulator/1(Vmes (pu))
  Product/1 -> N/1
  Constant/1 -> Voltage regulator/3(RegOn)
  Tap Changer Control/2(Ready) -> Voltage regulator/2(Ready)
  Voltage change per tap/1 -> Sum/2
  Constant5/1 -> Sum/1
  Voltage regulator/1(Up) -> Tap Changer Control/1("Up ")
  Tap Changer Control/1(TapNo) -> Voltage change per tap/1, Tap/1  "Tap"
  1/1 -> Product/2
  Sum/1 -> Product/1
  Voltage regulator/2(Down) -> Tap Changer Control/2("Down ")

== system IEEE13_DVR_DSTATCOM_PV_Wind/Regulator 1/Single Phase SVR_B/Line Drop Compensator ==
  note: Vm=Vsec-Isec(Rc+jXc)
  Isec : Inport
  Vsec : Inport  Port=2
  "        " : spsLinearTransformerLib/Linear Transformer  UNITS=SI  NominalPower=[pNom fNom]  winding1=[vNom/ptRatio 1e-7 1e-8]  winding2=[vNom/ptRatio 1e-7 1e-8]  ThreeWindings=off  winding3=[3.15e+005 0.7938 0.084225]  RmLm=[1e5 1e5]  Measurements=None  DataType=on
  "CTS  " : spsControlledCurrentSourceLib/Controlled Current Source  Initialize=on  Source_Type=AC  Amplitude=0  Phase=0  Frequency=0  Measurements=None
  "PTS  " : spsControlledVoltageSourceLib/Controlled Voltage Source  Initialize=on  Source_Type=AC  Amplitude=0  Phase=0  Frequency=0  Measurements=None
  RMS : spsRMSLib/RMS  TrueRMS=on  Freq=60  RMSInit=120  Ts=0
  Raux : spsSeriesRLCBranchLib/Series RLC Branch  LConnTagsString=__new0  RConnTagsString=__new0  BranchType=R  Resistance=1e3  Inductance=1.6 / (120*pi)  SetiL0=off  InitialCurrent=0  Capacitance=1e-6  Setx0=off  InitialVoltage=0  Measurements=None
  Rc+jXc : spsSeriesRLCBranchLib/Series RLC Branch  LConnTagsString=__new0  RConnTagsString=__new0  BranchType=RL  Resistance=Rc  Inductance=Xc / (2*pi*fNom)  SetiL0=off  InitialCurrent=0  Capacitance=1e-6  Setx0=off  InitialVoltage=0  Measurements=None
  VRelay : spsVoltageMeasurementLib/Voltage Measurement  PhasorSimulation=off  OutputType=Complex  PSBequivalent=0
  Vm : Outport
  wires:
  Vsec/1 -> "PTS  "/1
  Isec/1 -> "CTS  "/1
  VRelay/1 -> RMS/1
  RMS/1 -> Vm/1
  connections:
  VRelay/LConn2 -- "PTS  "/LConn1
  "        "/LConn2 -- "CTS  "/LConn1 -- Raux/RConn1 -- Rc+jXc/RConn1
  "CTS  "/RConn1 -- "        "/LConn1 -- Rc+jXc/LConn1 -- Raux/LConn1
  "        "/RConn2 -- VRelay/LConn1
  "PTS  "/RConn1 -- "        "/RConn1

== system IEEE13_DVR_DSTATCOM_PV_Wind/Regulator 1/Single Phase SVR_B/Transformer with Taps ==
  note: Isec on CT Ratio base
  note: Vsec on Pt Ratio base
  N : Inport
  "    " : Gain  Gain=1/ptRatio
  " 1" : Gain  Gain=1/ctRatio
  CT : spsCurrentMeasurementLib/Current Measurement  PhasorSimulation=off  OutputType=Complex  PSBequivalent=0
  Ground1 : spsGroundLib/Ground  LConnTagsString=a
  Ground2 : spsGroundLib/Ground  LConnTagsString=a
  Ground3 : spsGroundLib/Ground  LConnTagsString=a
  Memory : Memory
  Memory1 : Memory
  PT : spsVoltageMeasurementLib/Voltage Measurement  PhasorSimulation=off  OutputType=Complex  PSBequivalent=0
  "Variable-Ratio Transformer " : spsVariableRatioTransformerLib/Variable-Ratio Transformer
  rs : spsSeriesRLCBranchLib/Series RLC Branch  LConnTagsString=__new0  RConnTagsString=__new0  BranchType=R  Resistance=1e-6  Inductance=1e-3  SetiL0=off  InitialCurrent=0  Capacitance=1e-6  Setx0=off  InitialVoltage=0  Measurements=None
  L : PMIOPort  Tag=PMCPort  Side=Right
  S : PMIOPort  Port=2  Side=Left
  Isec : Outport
  Vsec : Outport  Port=2
  wires:
  Memory/1 -> Isec/1
  Memory1/1 -> Vsec/1
  N/1 -> "Variable-Ratio Transformer "/1
  " 1"/1 -> Memory/1
  CT/1 -> " 1"/1
  PT/1 -> "    "/1
  "    "/1 -> Memory1/1
  connections:
  S/RConn1 -- "Variable-Ratio Transformer "/LConn1
  Ground2/LConn1 -- "Variable-Ratio Transformer "/RConn2
  Ground3/LConn1 -- "Variable-Ratio Transformer "/LConn2
  "Variable-Ratio Transformer "/RConn1 -- rs/LConn1
  CT/RConn1 -- L/RConn1
  PT/LConn1 -- CT/LConn1 -- rs/RConn1
  PT/LConn2 -- Ground1/LConn1
